simulink model "balance_car_lqi"  (R2025b)
settings: Solver=ode15s  StartTime=0.0  StopTime=18  MaxStep=.001  RelTol=1e-5  AbsTol=1e-7
PostLoadFcn:
  | addpath(fileparts(fileparts(get_param(bdroot,'FileName'))));p=balance_setup;addpath(fullfile(p.root,'模型','仿真模型','通用URDF','meshes'));
model workspace (MAT data in the model file):
  suite_config = [7 2 0.00156420808869 -26.9746825695 -2.51185819954e-13 -15.7931791592 2.23675238355e-14 -22.0753502191 4.70720143585e-15 -1.84256370574 1.59828709082e-15 1.91428022169e-14 ... (41 elements, 1x41)]
  terrain_dimensions = [0.613404356919  0.35  0.02; 0.2  0.35  0.02; 0.613404356919  0.35  0.02; 0.04  0.06  0.02]
  terrain_on = 0
  terrain_rotation_deg = [-12; 0; 12; 0]
  terrain_translation = [0.552079116908  0  0.0539854924937; 0.95  0  0.117533937002; 1.34792088309  0  0.0539854924937; 1.82  0.0662682  -0.007]
values from neighbouring files (symbols this model uses):
  m = max(1,round(taus(k)/dt))    [analyze_imu_stationary.m]    (also in compare_encoder_ab.m = replay.t>=10&replay.t<=10.7; design_encoder_ab.m = motor==side; design_imu.m = max(1,round(periods(k)/dt)); plot_dynamic_comparison.m = T.time_s>=0&T.time_s<=65)
  N = round(duration/h)+1    [compare_encoder_ab.m]    (also in screen_imu_lqi.m = ceil(count/5); simulate_lqi.m = round(options.duration/Ts)+1)
  s = jsondecode(fileread(fullfile(root,'esp32','lqi_firmware','selected_lqi.json')))    [compare_encoder_ab.m]    (also in design_encoder_ab.m = jsondecode(fileread(fullfile(root,'esp32','lqi_firmware','se; hardware_lqi_design.m = jsondecode(fileread(fullfile(fw,'selected_lqi.json'))); screen_common_notch.m; screen_imu_lqi.m = amp*(10*u^3-15*u^4+6*u^5))
  X = [T.distance T.speed pitch T.pitch_rate T.yaw T.yaw_rate T.velocity_integral T.yaw_integral]    [prepare_online_lqi.m]    (also in screen_imu_lqi.m = X(1:k,:); simulate_lqi.m = X(1:k,:))
  Z = [theta(1:end-h),q(1:end-h),u(1:end-h),ones(n-h,1)]    [prepare_online_lqi.m]
undefined symbols (not defined in the file or in its folder): Y
libraries: sm_lib x48, nesl_utility x27
(part 2 of 2)

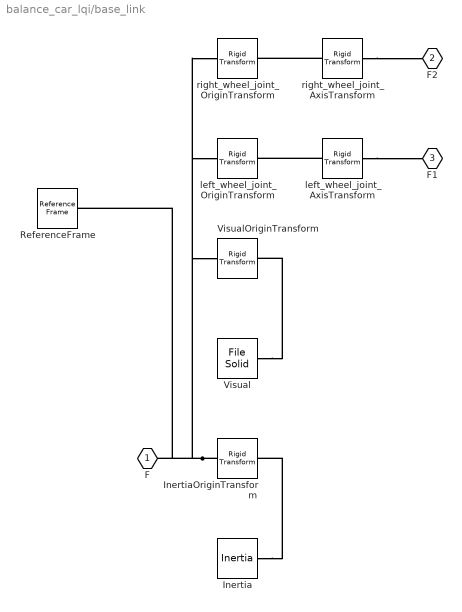
== system balance_car_lqi/base_link ==
  Inertia : sm_lib/Body Elements/Inertia  InertiaType=Custom  Mass=0.2771  MassUnits=kg  CenterOfMass=[0, 0, 0]  CenterOfMassUnits=m  MomentsOfInertia=[0.0006191390109428378, 0.000311847668361045, 0.000388176637385571]  MomentsOfInertiaUnits=kg*m^2  ProductsOfInertia=[-1.767576624229698e-07, -3.850274462317628e-08, 2.823397326959528e-07]  ProductsOfInertiaUnits=kg*m^2  GraphicType=None  MarkerShape=Inertia  MarkerSize=20  GraphicVisPropType=SimpleVisualProperties  GraphicDiffuseColor=[0.5 0.5 0.5]  GraphicOpacity=1  GraphicSpecularColor=[0.5 0.5 0.5 1.0]  GraphicAmbientColor=[0.15 0.15 0.15 1.0]  GraphicEmissiveColor=[0.0 0.0 0.0 1.0]  GraphicShininess=75
  InertiaOriginTransform : sm_lib/Frames and Transforms/Rigid Transform  RotationMethod=RotationSequence  FollAlignAxisA=+X  BaseAlignAxisA=+Y  FollAlignAxisB=+Y  BaseAlignAxisB=+Z  RotationStandardAxis=+Z  RotationAngle=0  RotationAngleUnits=deg  RotationArbitraryAxis=[0 0 1]  RotationSequenceAxes=BaseAxes  RotationSequence=XYZ  RotationSequenceAngles=[0, 0, 0]  RotationSequenceAnglesUnits=rad  RotationMatrix=[1 0 0;0 1 0;0 0 1]  Quaternion=[1 0 0 0]  TranslationMethod=Cartesian  TranslationCartesianOffset=[-5.71393596063e-05, -4.53146929236e-05, 0.0365292274203]  TranslationCartesianOffsetUnits=m  TranslationStandardAxis=+Z  TranslationStandardOffset=0  TranslationStandardOffsetUnits=m  TranslationROffset=0  TranslationROffsetUnits=m  TranslationThetaOffset=0  TranslationThetaOffsetUnits=deg  TranslationZOffset=0  TranslationZOffsetUnits=m
  ReferenceFrame : sm_lib/Frames and Transforms/Reference Frame
  Visual : sm_lib/Body Elements/File Solid  ExtGeomFileName=body.stl  UnitType=Custom  ExtGeomFileUnits=m  StepReaderType=HEX  ExportConvexHullGeometry=off  InertiaType=Custom  BasedOnType=DensityFromFile  Density=1000  DensityUnits=kg/m^3  Mass=0  MassUnits=kg  CenterOfMass=[0, 0, 0]  CenterOfMassUnits=m  MomentsOfInertia=[0, 0, 0]  MomentsOfInertiaUnits=kg*m^2  ProductsOfInertia=[0, 0, 0]  ProductsOfInertiaUnits=kg*m^2  GraphicType=FromGeometry  MarkerShape=Sphere  MarkerSize=10  GraphicVisPropType=SimpleVisualProperties  GraphicDiffuseColor=[0.12, 0.4, 0.65]  GraphicOpacity=1  GraphicSpecularColor=[0.5 0.5 0.5 1.0]  GraphicAmbientColor=[0.15 0.15 0.15 1.0]  GraphicEmissiveColor=[0.0 0.0 0.0 1.0]  GraphicShininess=75  DoExposeReferenceFrame=on  SerializedFrames=<Frames/>
  VisualOriginTransform : sm_lib/Frames and Transforms/Rigid Transform  RotationMethod=RotationSequence  FollAlignAxisA=+X  BaseAlignAxisA=+Y  FollAlignAxisB=+Y  BaseAlignAxisB=+Z  RotationStandardAxis=+Z  RotationAngle=0  RotationAngleUnits=deg  RotationArbitraryAxis=[0 0 1]  RotationSequenceAxes=BaseAxes  RotationSequence=XYZ  RotationSequenceAngles=[0, 0, 0]  RotationSequenceAnglesUnits=rad  RotationMatrix=[1 0 0;0 1 0;0 0 1]  Quaternion=[1 0 0 0]  TranslationMethod=Cartesian  TranslationCartesianOffset=[0, 0, 0]  TranslationCartesianOffsetUnits=m  TranslationStandardAxis=+Z  TranslationStandardOffset=0  TranslationStandardOffsetUnits=m  TranslationROffset=0  TranslationROffsetUnits=m  TranslationThetaOffset=0  TranslationThetaOffsetUnits=deg  TranslationZOffset=0  TranslationZOffsetUnits=m
  left_wheel_joint_AxisTransform : sm_lib/Frames and Transforms/Rigid Transform  RotationMethod=ArbitraryAxis  FollAlignAxisA=+X  BaseAlignAxisA=+Y  FollAlignAxisB=+Y  BaseAlignAxisB=+Z  RotationStandardAxis=+Z  RotationAngle=1.570796326794897  RotationAngleUnits=rad  RotationArbitraryAxis=[-1, 0, 0]  RotationSequenceAxes=FollowerAxes  RotationSequence=XYX  RotationSequenceAngles=[0 0 0]  RotationSequenceAnglesUnits=deg  RotationMatrix=[1 0 0;0 1 0;0 0 1]  Quaternion=[1 0 0 0]  TranslationMethod=Cartesian  TranslationCartesianOffset=[0, 0, 0]  TranslationCartesianOffsetUnits=m  TranslationStandardAxis=+Z  TranslationStandardOffset=0  TranslationStandardOffsetUnits=m  TranslationROffset=0  TranslationROffsetUnits=m  TranslationThetaOffset=0  TranslationThetaOffsetUnits=deg  TranslationZOffset=0  TranslationZOffsetUnits=m
  left_wheel_joint_OriginTransform : sm_lib/Frames and Transforms/Rigid Transform  RotationMethod=RotationSequence  FollAlignAxisA=+X  BaseAlignAxisA=+Y  FollAlignAxisB=+Y  BaseAlignAxisB=+Z  RotationStandardAxis=+Z  RotationAngle=0  RotationAngleUnits=deg  RotationArbitraryAxis=[0 0 1]  RotationSequenceAxes=BaseAxes  RotationSequence=XYZ  RotationSequenceAngles=[0, 0, 0]  RotationSequenceAnglesUnits=rad  RotationMatrix=[1 0 0;0 1 0;0 0 1]  Quaternion=[1 0 0 0]  TranslationMethod=Cartesian  TranslationCartesianOffset=[0, 0.0662682, 0]  TranslationCartesianOffsetUnits=m  TranslationStandardAxis=+Z  TranslationStandardOffset=0  TranslationStandardOffsetUnits=m  TranslationROffset=0  TranslationROffsetUnits=m  TranslationThetaOffset=0  TranslationThetaOffsetUnits=deg  TranslationZOffset=0  TranslationZOffsetUnits=m
  right_wheel_joint_AxisTransform : sm_lib/Frames and Transforms/Rigid Transform  RotationMethod=ArbitraryAxis  FollAlignAxisA=+X  BaseAlignAxisA=+Y  FollAlignAxisB=+Y  BaseAlignAxisB=+Z  RotationStandardAxis=+Z  RotationAngle=1.570796326794897  RotationAngleUnits=rad  RotationArbitraryAxis=[-1, 0, 0]  RotationSequenceAxes=FollowerAxes  RotationSequence=XYX  RotationSequenceAngles=[0 0 0]  RotationSequenceAnglesUnits=deg  RotationMatrix=[1 0 0;0 1 0;0 0 1]  Quaternion=[1 0 0 0]  TranslationMethod=Cartesian  TranslationCartesianOffset=[0, 0, 0]  TranslationCartesianOffsetUnits=m  TranslationStandardAxis=+Z  TranslationStandardOffset=0  TranslationStandardOffsetUnits=m  TranslationROffset=0  TranslationROffsetUnits=m  TranslationThetaOffset=0  TranslationThetaOffsetUnits=deg  TranslationZOffset=0  TranslationZOffsetUnits=m
  right_wheel_joint_OriginTransform : sm_lib/Frames and Transforms/Rigid Transform  RotationMethod=RotationSequence  FollAlignAxisA=+X  BaseAlignAxisA=+Y  FollAlignAxisB=+Y  BaseAlignAxisB=+Z  RotationStandardAxis=+Z  RotationAngle=0  RotationAngleUnits=deg  RotationArbitraryAxis=[0 0 1]  RotationSequenceAxes=BaseAxes  RotationSequence=XYZ  RotationSequenceAngles=[0, 0, 0]  RotationSequenceAnglesUnits=rad  RotationMatrix=[1 0 0;0 1 0;0 0 1]  Quaternion=[1 0 0 0]  TranslationMethod=Cartesian  TranslationCartesianOffset=[0, -0.0662682, 0]  TranslationCartesianOffsetUnits=m  TranslationStandardAxis=+Z  TranslationStandardOffset=0  TranslationStandardOffsetUnits=m  TranslationROffset=0  TranslationROffsetUnits=m  TranslationThetaOffset=0  TranslationThetaOffsetUnits=deg  TranslationZOffset=0  TranslationZOffsetUnits=m
  F : PMIOPort  Side=Left
  F2 : PMIOPort  Port=2  Side=Right
  F1 : PMIOPort  Port=3  Side=Right
  connections:
  Inertia/RConn1 -- InertiaOriginTransform/RConn1
  ReferenceFrame/RConn1 -- InertiaOriginTransform/LConn1 -- VisualOriginTransform/LConn1 -- left_wheel_joint_OriginTransform/LConn1 -- right_wheel_joint_OriginTransform/LConn1 -- F/RConn1
  Visual/RConn1 -- VisualOriginTransform/RConn1
  left_wheel_joint_AxisTransform/RConn1 -- F1/RConn1
  left_wheel_joint_AxisTransform/LConn1 -- left_wheel_joint_OriginTransform/RConn1
  right_wheel_joint_AxisTransform/RConn1 -- F2/RConn1
  right_wheel_joint_AxisTransform/LConn1 -- right_wheel_joint_OriginTransform/RConn1

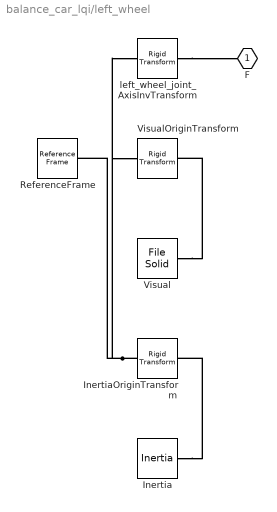
== system balance_car_lqi/left_wheel ==
  Inertia : sm_lib/Body Elements/Inertia  InertiaType=Custom  Mass=0.06270000000000001  MassUnits=kg  CenterOfMass=[0, 0, 0]  CenterOfMassUnits=m  MomentsOfInertia=[1.917831991019924e-05, 2.996788998409583e-05, 1.917831830082714e-05]  MomentsOfInertiaUnits=kg*m^2  ProductsOfInertia=[1.265848450812081e-12, -7.252640958073256e-12, 3.83369315636605e-12]  ProductsOfInertiaUnits=kg*m^2  GraphicType=None  MarkerShape=Inertia  MarkerSize=20  GraphicVisPropType=SimpleVisualProperties  GraphicDiffuseColor=[0.5 0.5 0.5]  GraphicOpacity=1  GraphicSpecularColor=[0.5 0.5 0.5 1.0]  GraphicAmbientColor=[0.15 0.15 0.15 1.0]  GraphicEmissiveColor=[0.0 0.0 0.0 1.0]  GraphicShininess=75
  InertiaOriginTransform : sm_lib/Frames and Transforms/Rigid Transform  RotationMethod=RotationSequence  FollAlignAxisA=+X  BaseAlignAxisA=+Y  FollAlignAxisB=+Y  BaseAlignAxisB=+Z  RotationStandardAxis=+Z  RotationAngle=0  RotationAngleUnits=deg  RotationArbitraryAxis=[0 0 1]  RotationSequenceAxes=BaseAxes  RotationSequence=XYZ  RotationSequenceAngles=[0, 0, 0]  RotationSequenceAnglesUnits=rad  RotationMatrix=[1 0 0;0 1 0;0 0 1]  Quaternion=[1 0 0 0]  TranslationMethod=Cartesian  TranslationCartesianOffset=[3.60871449673e-09, -0.00137780420767, -5.37617755869e-09]  TranslationCartesianOffsetUnits=m  TranslationStandardAxis=+Z  TranslationStandardOffset=0  TranslationStandardOffsetUnits=m  TranslationROffset=0  TranslationROffsetUnits=m  TranslationThetaOffset=0  TranslationThetaOffsetUnits=deg  TranslationZOffset=0  TranslationZOffsetUnits=m
  ReferenceFrame : sm_lib/Frames and Transforms/Reference Frame
  Visual : sm_lib/Body Elements/File Solid  ExtGeomFileName=left_wheel.stl  UnitType=Custom  ExtGeomFileUnits=m  StepReaderType=HEX  ExportConvexHullGeometry=off  InertiaType=Custom  BasedOnType=DensityFromFile  Density=1000  DensityUnits=kg/m^3  Mass=0  MassUnits=kg  CenterOfMass=[0, 0, 0]  CenterOfMassUnits=m  MomentsOfInertia=[0, 0, 0]  MomentsOfInertiaUnits=kg*m^2  ProductsOfInertia=[0, 0, 0]  ProductsOfInertiaUnits=kg*m^2  GraphicType=FromGeometry  MarkerShape=Sphere  MarkerSize=10  GraphicVisPropType=SimpleVisualProperties  GraphicDiffuseColor=[0.16, 0.18, 0.16]  GraphicOpacity=1  GraphicSpecularColor=[0.5 0.5 0.5 1.0]  GraphicAmbientColor=[0.15 0.15 0.15 1.0]  GraphicEmissiveColor=[0.0 0.0 0.0 1.0]  GraphicShininess=75  DoExposeReferenceFrame=on  SerializedFrames=<Frames/>
  VisualOriginTransform : sm_lib/Frames and Transforms/Rigid Transform  RotationMethod=RotationSequence  FollAlignAxisA=+X  BaseAlignAxisA=+Y  FollAlignAxisB=+Y  BaseAlignAxisB=+Z  RotationStandardAxis=+Z  RotationAngle=0  RotationAngleUnits=deg  RotationArbitraryAxis=[0 0 1]  RotationSequenceAxes=BaseAxes  RotationSequence=XYZ  RotationSequenceAngles=[0, 0, 0]  RotationSequenceAnglesUnits=rad  RotationMatrix=[1 0 0;0 1 0;0 0 1]  Quaternion=[1 0 0 0]  TranslationMethod=Cartesian  TranslationCartesianOffset=[0, 0, 0]  TranslationCartesianOffsetUnits=m  TranslationStandardAxis=+Z  TranslationStandardOffset=0  TranslationStandardOffsetUnits=m  TranslationROffset=0  TranslationROffsetUnits=m  TranslationThetaOffset=0  TranslationThetaOffsetUnits=deg  TranslationZOffset=0  TranslationZOffsetUnits=m
  left_wheel_joint_AxisInvTransform : sm_lib/Frames and Transforms/Rigid Transform  RotationMethod=ArbitraryAxis  FollAlignAxisA=+X  BaseAlignAxisA=+Y  FollAlignAxisB=+Y  BaseAlignAxisB=+Z  RotationStandardAxis=+Z  RotationAngle=1.570796326794897  RotationAngleUnits=rad  RotationArbitraryAxis=[-1, 0, 0]  RotationSequenceAxes=FollowerAxes  RotationSequence=XYX  RotationSequenceAngles=[0 0 0]  RotationSequenceAnglesUnits=deg  RotationMatrix=[1 0 0;0 1 0;0 0 1]  Quaternion=[1 0 0 0]  TranslationMethod=Cartesian  TranslationCartesianOffset=[0, 0, 0]  TranslationCartesianOffsetUnits=m  TranslationStandardAxis=+Z  TranslationStandardOffset=0  TranslationStandardOffsetUnits=m  TranslationROffset=0  TranslationROffsetUnits=m  TranslationThetaOffset=0  TranslationThetaOffsetUnits=deg  TranslationZOffset=0  TranslationZOffsetUnits=m
  F : PMIOPort  Side=Left
  connections:
  Inertia/RConn1 -- InertiaOriginTransform/RConn1
  ReferenceFrame/RConn1 -- InertiaOriginTransform/LConn1 -- VisualOriginTransform/LConn1 -- left_wheel_joint_AxisInvTransform/LConn1
  Visual/RConn1 -- VisualOriginTransform/RConn1
  left_wheel_joint_AxisInvTransform/RConn1 -- F/RConn1

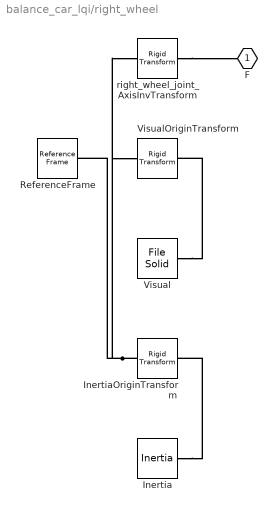
== system balance_car_lqi/right_wheel ==
  Inertia : sm_lib/Body Elements/Inertia  InertiaType=Custom  Mass=0.06270000000000001  MassUnits=kg  CenterOfMass=[0, 0, 0]  CenterOfMassUnits=m  MomentsOfInertia=[1.917831991019923e-05, 2.996788998409583e-05, 1.917831830082714e-05]  MomentsOfInertiaUnits=kg*m^2  ProductsOfInertia=[-1.265848447928984e-12, 7.252640957165455e-12, 3.833693155565584e-12]  ProductsOfInertiaUnits=kg*m^2  GraphicType=None  MarkerShape=Inertia  MarkerSize=20  GraphicVisPropType=SimpleVisualProperties  GraphicDiffuseColor=[0.5 0.5 0.5]  GraphicOpacity=1  GraphicSpecularColor=[0.5 0.5 0.5 1.0]  GraphicAmbientColor=[0.15 0.15 0.15 1.0]  GraphicEmissiveColor=[0.0 0.0 0.0 1.0]  GraphicShininess=75
  InertiaOriginTransform : sm_lib/Frames and Transforms/Rigid Transform  RotationMethod=RotationSequence  FollAlignAxisA=+X  BaseAlignAxisA=+Y  FollAlignAxisB=+Y  BaseAlignAxisB=+Z  RotationStandardAxis=+Z  RotationAngle=0  RotationAngleUnits=deg  RotationArbitraryAxis=[0 0 1]  RotationSequenceAxes=BaseAxes  RotationSequence=XYZ  RotationSequenceAngles=[0, 0, 0]  RotationSequenceAnglesUnits=rad  RotationMatrix=[1 0 0;0 1 0;0 0 1]  Quaternion=[1 0 0 0]  TranslationMethod=Cartesian  TranslationCartesianOffset=[-3.60871449808e-09, 0.00137780420767, -5.37617755869e-09]  TranslationCartesianOffsetUnits=m  TranslationStandardAxis=+Z  TranslationStandardOffset=0  TranslationStandardOffsetUnits=m  TranslationROffset=0  TranslationROffsetUnits=m  TranslationThetaOffset=0  TranslationThetaOffsetUnits=deg  TranslationZOffset=0  TranslationZOffsetUnits=m
  ReferenceFrame : sm_lib/Frames and Transforms/Reference Frame
  Visual : sm_lib/Body Elements/File Solid  ExtGeomFileName=right_wheel.stl  UnitType=Custom  ExtGeomFileUnits=m  StepReaderType=HEX  ExportConvexHullGeometry=off  InertiaType=Custom  BasedOnType=DensityFromFile  Density=1000  DensityUnits=kg/m^3  Mass=0  MassUnits=kg  CenterOfMass=[0, 0, 0]  CenterOfMassUnits=m  MomentsOfInertia=[0, 0, 0]  MomentsOfInertiaUnits=kg*m^2  ProductsOfInertia=[0, 0, 0]  ProductsOfInertiaUnits=kg*m^2  GraphicType=FromGeometry  MarkerShape=Sphere  MarkerSize=10  GraphicVisPropType=SimpleVisualProperties  GraphicDiffuseColor=[0.16, 0.18, 0.16]  GraphicOpacity=1  GraphicSpecularColor=[0.5 0.5 0.5 1.0]  GraphicAmbientColor=[0.15 0.15 0.15 1.0]  GraphicEmissiveColor=[0.0 0.0 0.0 1.0]  GraphicShininess=75  DoExposeReferenceFrame=on  SerializedFrames=<Frames/>
  VisualOriginTransform : sm_lib/Frames and Transforms/Rigid Transform  RotationMethod=RotationSequence  FollAlignAxisA=+X  BaseAlignAxisA=+Y  FollAlignAxisB=+Y  BaseAlignAxisB=+Z  RotationStandardAxis=+Z  RotationAngle=0  RotationAngleUnits=deg  RotationArbitraryAxis=[0 0 1]  RotationSequenceAxes=BaseAxes  RotationSequence=XYZ  RotationSequenceAngles=[0, 0, 0]  RotationSequenceAnglesUnits=rad  RotationMatrix=[1 0 0;0 1 0;0 0 1]  Quaternion=[1 0 0 0]  TranslationMethod=Cartesian  TranslationCartesianOffset=[0, 0, 0]  TranslationCartesianOffsetUnits=m  TranslationStandardAxis=+Z  TranslationStandardOffset=0  TranslationStandardOffsetUnits=m  TranslationROffset=0  TranslationROffsetUnits=m  TranslationThetaOffset=0  TranslationThetaOffsetUnits=deg  TranslationZOffset=0  TranslationZOffsetUnits=m
  right_wheel_joint_AxisInvTransform : sm_lib/Frames and Transforms/Rigid Transform  RotationMethod=ArbitraryAxis  FollAlignAxisA=+X  BaseAlignAxisA=+Y  FollAlignAxisB=+Y  BaseAlignAxisB=+Z  RotationStandardAxis=+Z  RotationAngle=1.570796326794897  RotationAngleUnits=rad  RotationArbitraryAxis=[-1, 0, 0]  RotationSequenceAxes=FollowerAxes  RotationSequence=XYX  RotationSequenceAngles=[0 0 0]  RotationSequenceAnglesUnits=deg  RotationMatrix=[1 0 0;0 1 0;0 0 1]  Quaternion=[1 0 0 0]  TranslationMethod=Cartesian  TranslationCartesianOffset=[0, 0, 0]  TranslationCartesianOffsetUnits=m  TranslationStandardAxis=+Z  TranslationStandardOffset=0  TranslationStandardOffsetUnits=m  TranslationROffset=0  TranslationROffsetUnits=m  TranslationThetaOffset=0  TranslationThetaOffsetUnits=deg  TranslationZOffset=0  TranslationZOffsetUnits=m
  F : PMIOPort  Side=Left
  connections:
  Inertia/RConn1 -- InertiaOriginTransform/RConn1
  ReferenceFrame/RConn1 -- InertiaOriginTransform/LConn1 -- VisualOriginTransform/LConn1 -- right_wheel_joint_AxisInvTransform/LConn1
  Visual/RConn1 -- VisualOriginTransform/RConn1
  right_wheel_joint_AxisInvTransform/RConn1 -- F/RConn1

== matlab function balance_car_lqi/Balance_Controller ==
  data: raw input; out output; cfg input
function out=balance_suite_controller(raw,cfg)
%#codegen
% raw=[time x vx y vy z vz qw qx qy qz wx wy wz]，角速度在世界坐标。
% out=[实际tau(2) state(6) ref(6) force(3) torque(3) fall 执行指令(2) PID目标(2)]。
% cfg(16)=2时执行指令是iq/A；其余模式为转矩/Nm。
persistent distance prevV velocityIntegral pitchIntegral yawIntegral lqiIntegral
if isempty(distance)
 distance=0;prevV=0;velocityIntegral=0;pitchIntegral=0;yawIntegral=0;lqiIntegral=zeros(2,1);
end
t=raw(1); qw=raw(8);qx=raw(9);qy=raw(10);qz=raw(11);
R=[1-2*(qy^2+qz^2) 2*(qx*qy-qw*qz) 2*(qx*qz+qw*qy); ...
   2*(qx*qy+qw*qz) 1-2*(qx^2+qz^2) 2*(qy*qz-qw*qx); ...
   2*(qx*qz-qw*qy) 2*(qy*qz+qw*qx) 1-2*(qx^2+qy^2)];
pitch=atan2(-R(3,1),hypot(R(1,1),R(2,1)));yaw=atan2(R(2,1),R(1,1));
roll=atan2(R(3,2),R(3,3)); wb=R'*raw(12:14);
pitchRate=cos(roll)*wb(2)-sin(roll)*wb(3);
yawRate=(sin(roll)*wb(2)+cos(roll)*wb(3))/cos(pitch);
v=cos(yaw)*raw(3)+sin(yaw)*raw(5);
Ts=cfg(31);
if t>0,distance=distance+Ts*(prevV+v)/2;end
prevV=v;
state=[distance;v;pitch-cfg(3);pitchRate;yaw;yawRate];
ref=zeros(6,1);F=zeros(3,1);T=zeros(3,1);scenario=round(cfg(1));
fast=round(cfg(34))==1;
if scenario==2 % 指令行驶：0.3m前进，随后后退到0.1m。
 if fast
  [p1,v1]=smoothmove(t,1,1.2,.30);[p2,v2]=smoothmove(t,3.8,1.2,-.20);
 else
  [p1,v1]=smoothmove(t,1,3,.30);[p2,v2]=smoothmove(t,6,2,-.20);
 end
 ref(1)=p1+p2;ref(2)=v1+v2;
elseif scenario==3 % 原地转60°，随后返回20°。
 if fast
  [a,w]=smoothmove(t,1,1.2,pi/3);[a2,w2]=smoothmove(t,4,1.2,-2*pi/9);
 else
  [a,w]=smoothmove(t,1,2,pi/3);[a2,w2]=smoothmove(t,5,2,-2*pi/9);
 end
 ref(5)=a+a2;ref(6)=w+w2;
elseif scenario==4 % 向前运动同时转弯。
 if fast
  [s,vs]=smoothmove(t,1,3,.6);[a,w]=smoothmove(t,1.5,1.5,pi/3);
 else
  [s,vs]=smoothmove(t,1,6,.6);[a,w]=smoothmove(t,2,3,pi/3);
 end
 ref(1)=s;ref(2)=vs;ref(5)=a;ref(6)=w;
elseif scenario==5 % 轮轴处的外力及绕竖直轴的外转矩脉冲。
 if t>=2 && t<2.15,F(1)=.4;end
 if t>=4 && t<4.15,T(3)=.002;end
elseif scenario==6 % 地形路线：经过缓坡、平台、下坡和单侧小凸起。
 [s,vs]=smoothmove(t,1,8,.75);ref(1)=s;ref(2)=vs;
elseif scenario==7 % 恒定扰动：比较两种控制器的稳态误差。
 if t>=2,F(1)=.08;T(3)=.0004;end
elseif scenario==8 % 明显坡道：上坡、平台、下坡、单侧凸起。
 [s,vs]=smoothmove(t,1,20,cfg(36));ref(1)=s;ref(2)=vs;
elseif scenario==9 % 斜面中段停12秒，随后继续通过坡顶与下坡。
 [s1,v1]=smoothmove(t,1,6,cfg(35));
 [s2,v2]=smoothmove(t,19,11,cfg(36)-cfg(35));
 ref(1)=s1+s2;ref(2)=v1+v2;
end
error=state-ref;
pidTarget=zeros(2,1);
if cfg(16)<.5
 K=reshape(cfg(4:15),2,6);effort=-K*error;
elseif cfg(16)>2.5
 K=reshape(cfg(4:15),2,6);Ki=reshape(cfg(38:41),2,2);
 integralError=[error(1);atan2(sin(error(5)),cos(error(5)))];
 candidate=lqiIntegral+Ts*integralError;
 candidate=max(-[.3;1],min([.3;1],candidate));
 effort=-K*error-Ki*lqiIntegral;
 wheel=[(effort(1)-effort(2))/2;(effort(1)+effort(2))/2];
 if max(abs(wheel))<=cfg(2),lqiIntegral=candidate;end
else
 targetV=clamp(ref(2)+cfg(22)*(ref(1)-state(1)),cfg(23));
 velocityError=targetV-v;
 vi=clamp(velocityIntegral+Ts*velocityError,cfg(25));
 targetUnclamped=cfg(20)*velocityError+cfg(21)*vi;
 targetPitch=clamp(targetUnclamped,cfg(24));
 pitchError=state(3)-targetPitch;
 piCandidate=clamp(pitchIntegral+Ts*pitchError,cfg(26));
 yawError=atan2(sin(ref(5)-yaw),cos(ref(5)-yaw));
 yi=clamp(yawIntegral+Ts*yawError,cfg(30));
 effort=[cfg(17)*pitchError+cfg(18)*piCandidate+cfg(19)*pitchRate; ...
  cfg(27)*yawError+cfg(28)*yi+cfg(29)*(ref(6)-yawRate)];
 % 转矩或倾角饱和时冻结相关积分。
 if max(abs([(effort(1)-effort(2))/2;(effort(1)+effort(2))/2]))<=cfg(2)
  pitchIntegral=piCandidate;yawIntegral=yi;
  if abs(targetUnclamped)<=cfg(24),velocityIntegral=vi;end
 end
 pidTarget=[targetV;targetPitch];
end
% effort(1)=左右转矩和，effort(2)=右减左。
tau=[(effort(1)-effort(2))/2;(effort(1)+effort(2))/2];
limit=cfg(2);
command=max(-limit,min(limit,tau));
tau=command.*[cfg(32);cfg(33)]; % 显式列向量，避免Simulink向量方向推断差异
if cfg(16)>1.5
 tau=tau*cfg(37); % 理想电流跟踪；实际Kt=标称Kt×左右执行增益。
end
out=[tau;state;ref;F;T;double(abs(pitch)>pi/4 || abs(roll)>pi/6);command;pidTarget];
end

function y=clamp(x,limit)
y=max(-limit,min(limit,x));
end

function [p,v]=smoothmove(t,start,duration,amplitude)
u=max(0,min(1,(t-start)/duration));
p=amplitude*(10*u^3-15*u^4+6*u^5);
if t<=start || t>=start+duration,v=0;
else,v=amplitude*(30*u^2-60*u^3+30*u^4)/duration;end
end
